simulink model "LKA_Controller"  (R2026a)
settings: Solver=FixedStepDiscrete  StopTime=inf  FixedStep=LKA.Ts
undefined symbols (not defined in the file): DiscIntNeverNeededParam, LKA
libraries: simulink x6, sl_discontinuities x2
Description:
  | Lane Keeping Assist: lane perception (validation, centre fusion, Kalman tracker), supervisor FSM, lane departure warning, pure pursuit / Stanley 2025 / MPC lateral controllers, a_y and jerk limited curvature command, steering actuator manager, turning radius.
settings Model: Creator=rithv  LastModifiedBy=rithv
settings DebuggingCC: AlgebraicLoopMsg=error
settings ModelReferenceCC: ModelReferenceNumInstancesAllowed=Single
settings GRTTargetCC: SubcomponentCodeInterfacePackaging=Nonreusable function

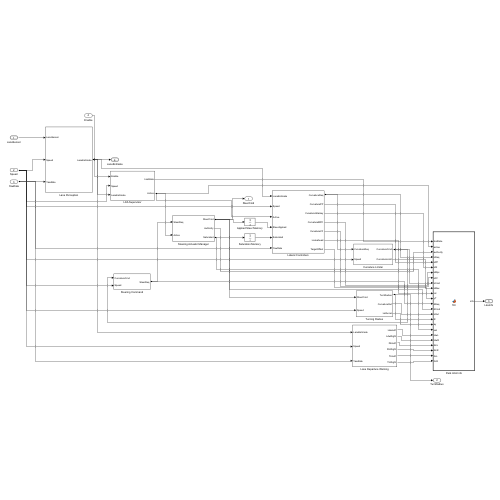
[thumbnail: Simulink's stored preview of the top-level diagram]
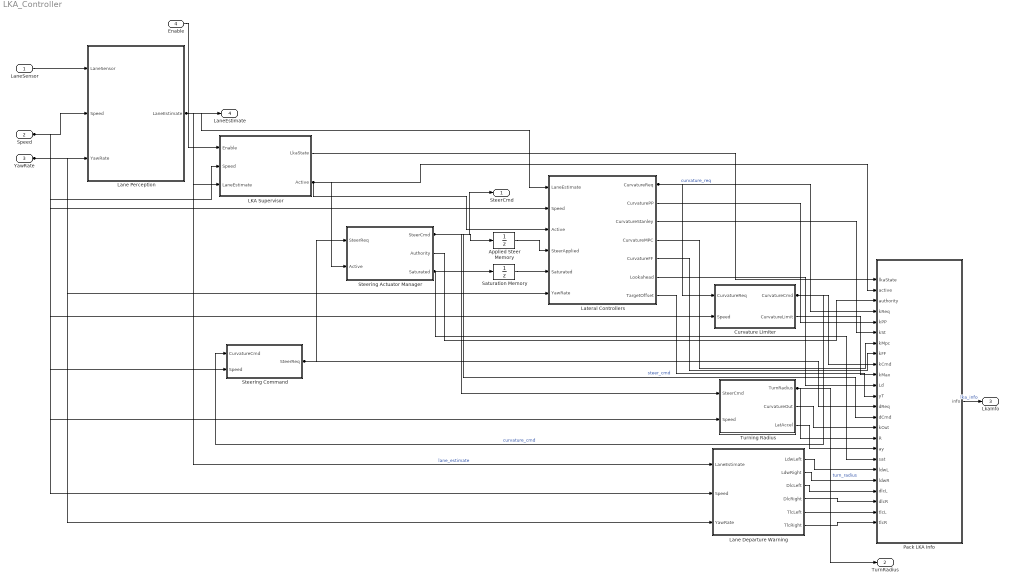
== system LKA_Controller ==
  LaneSensor : Inport  OutDataTypeStr=Bus: LaneSensorBus  SampleTime=LKA.Ts  BusOutputAsStruct=on
  Speed : Inport  Port=2  OutDataTypeStr=double  SampleTime=LKA.Ts
  YawRate : Inport  Port=3  OutDataTypeStr=double  SampleTime=LKA.Ts
  Enable : Inport  Port=4  OutDataTypeStr=boolean  SampleTime=LKA.Ts
  Applied Steer Memory : UnitDelay  SampleTime=-1
  Curvature Limiter : Subsystem
  LKA Supervisor : Subsystem
  Lane Departure Warning : Subsystem
  Lane Perception : Subsystem
  Lateral Controllers : Subsystem
  Pack LKA Info : MATLAB Function  TreatAsAtomicUnit=on
  Saturation Memory : UnitDelay  SampleTime=-1
  Steering Actuator Manager : Subsystem
  Steering Command : Subsystem
  Turning Radius : Subsystem
  SteerCmd : Outport  OutDataTypeStr=double
  TurnRadius : Outport  Port=2  OutDataTypeStr=double
  LkaInfo : Outport  Port=3  OutDataTypeStr=Bus: LkaInfoBus  BusOutputAsStruct=on
  LaneEstimate : Outport  Port=4  OutDataTypeStr=Bus: LaneEstimateBus  BusOutputAsStruct=on
  wires:
  Turning Radius/1(TurnRadius) -> TurnRadius/1, Pack LKA Info/16(R)  "turn_radius"
  Steering Command/1(SteerReq) -> Pack LKA Info/13(dReq), Steering Actuator Manager/1(SteerReq)
  Lane Departure Warning/2(LdwRight) -> Pack LKA Info/20(ldwR)
  LaneSensor/1 -> Lane Perception/1(LaneSensor)
  Steering Actuator Manager/1(SteerCmd) -> Turning Radius/1(SteerCmd), Pack LKA Info/14(dCmd), Applied Steer Memory/1, SteerCmd/1  "steer_cmd"
  Speed/1 -> LKA Supervisor/2(Speed), Lateral Controllers/2(Speed), Curvature Limiter/2(Speed), Steering Command/2(Speed), Turning Radius/2(Speed), Lane Perception/2(Speed), Lane Departure Warning/2(Speed)
  Enable/1 -> LKA Supervisor/1(Enable)
  Lane Departure Warning/5(TlcLeft) -> Pack LKA Info/23(tlcL)
  Lateral Controllers/5(CurvatureFF) -> Pack LKA Info/8(kFF)
  YawRate/1 -> Lateral Controllers/6(YawRate), Lane Perception/3(YawRate), Lane Departure Warning/3(YawRate)
  Lateral Controllers/2(CurvaturePP) -> Pack LKA Info/5(kPP)
  Saturation Memory/1 -> Lateral Controllers/5(Saturated)
  LKA Supervisor/1(LkaState) -> Pack LKA Info/1(lkaState)
  Lane Perception/1(LaneEstimate) -> Lateral Controllers/1(LaneEstimate), LKA Supervisor/3(LaneEstimate), LaneEstimate/1, Lane Departure Warning/1(LaneEstimate)  "lane_estimate"
  LKA Supervisor/2(Active) -> Lateral Controllers/3(Active), Pack LKA Info/2(active), Steering Actuator Manager/2(Active)
  Steering Actuator Manager/2(Authority) -> Pack LKA Info/3(authority)
  Steering Actuator Manager/3(Saturated) -> Pack LKA Info/18(sat), Saturation Memory/1
  Applied Steer Memory/1 -> Lateral Controllers/4(SteerApplied)
  Lateral Controllers/1(CurvatureReq) -> Curvature Limiter/1(CurvatureReq), Pack LKA Info/4(kReq)  "curvature_req"
  Lateral Controllers/3(CurvatureStanley) -> Pack LKA Info/6(kSt)
  Lateral Controllers/4(CurvatureMPC) -> Pack LKA Info/7(kMpc)
  Lateral Controllers/6(Lookahead) -> Pack LKA Info/11(Ld)
  Lateral Controllers/7(TargetOffset) -> Pack LKA Info/12(yT)
  Curvature Limiter/1(CurvatureCmd) -> Steering Command/1(CurvatureCmd), Pack LKA Info/9(kCmd)  "curvature_cmd"
  Curvature Limiter/2(CurvatureLimit) -> Pack LKA Info/10(kMax)
  Turning Radius/2(CurvatureOut) -> Pack LKA Info/15(kOut)
  Turning Radius/3(LatAccel) -> Pack LKA Info/17(ay)
  Lane Departure Warning/6(TlcRight) -> Pack LKA Info/24(tlcR)
  Lane Departure Warning/1(LdwLeft) -> Pack LKA Info/19(ldwL)
  Lane Departure Warning/3(DlcLeft) -> Pack LKA Info/21(dlcL)
  Lane Departure Warning/4(DlcRight) -> Pack LKA Info/22(dlcR)
  Pack LKA Info/1(info) -> LkaInfo/1  "lka_info"

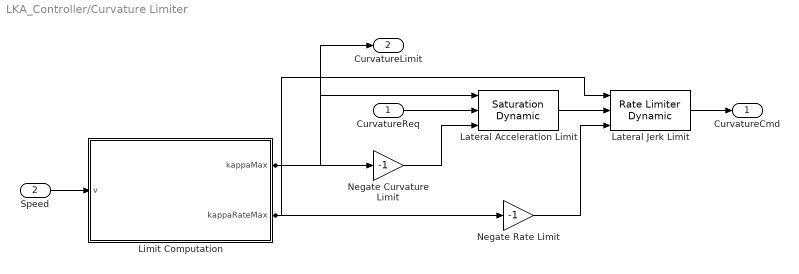
== system LKA_Controller/Curvature Limiter ==
  CurvatureReq : Inport
  Speed : Inport  Port=2
  Lateral Acceleration Limit : sl_discontinuities/Saturation Dynamic  OutMin=[]  OutMax=[]  OutDataTypeStr=Inherit: Same as second input  OutDataType=fixdt(1, 16)  OutScaling=2^-10  DoSatur=off
      settings: LibrarySourceBlock=|
      | simulink/Discontinuities/Saturation
      | Dynamic
  Lateral Jerk Limit : sl_discontinuities/Rate Limiter Dynamic
      settings: LibrarySourceBlock=|
      | simulink/Discontinuities/Rate Limiter
      | Dynamic
  Limit Computation : MATLAB Function  TreatAsAtomicUnit=on
  Negate Curvature Limit : Gain  Gain=-1
  Negate Rate Limit : Gain  Gain=-1
  CurvatureCmd : Outport
  CurvatureLimit : Outport  Port=2
  wires:
  Lateral Acceleration Limit/1 -> Lateral Jerk Limit/2
  Speed/1 -> Limit Computation/1(v)
  Negate Rate Limit/1 -> Lateral Jerk Limit/3
  CurvatureReq/1 -> Lateral Acceleration Limit/2
  Limit Computation/1(kappaMax) -> Negate Curvature Limit/1, Lateral Acceleration Limit/1, CurvatureLimit/1
  Limit Computation/2(kappaRateMax) -> Lateral Jerk Limit/1, Negate Rate Limit/1
  Lateral Jerk Limit/1 -> CurvatureCmd/1
  Negate Curvature Limit/1 -> Lateral Acceleration Limit/3

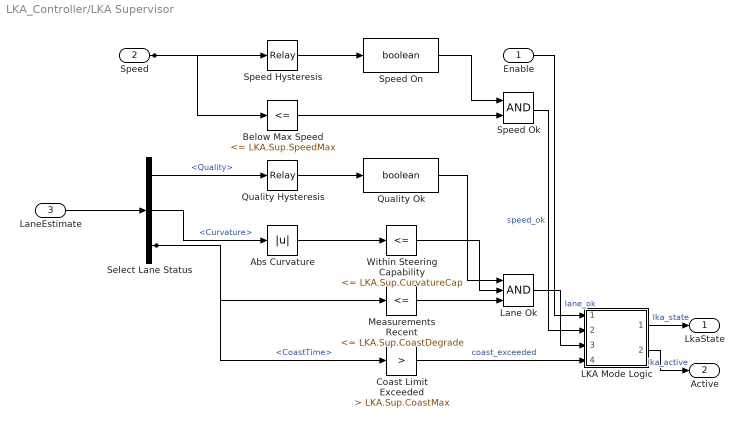
== system LKA_Controller/LKA Supervisor ==
  Enable : Inport
  Speed : Inport  Port=2
  LaneEstimate : Inport  Port=3
  Abs Curvature : Abs  SaturateOnIntegerOverflow=off
  Below Max Speed : simulink/Logic and Bit Operations/Compare To Constant  relop=<=  const=LKA.Sup.SpeedMax  OutDataTypeStr=boolean
  Coast Limit Exceeded : simulink/Logic and Bit Operations/Compare To Constant  relop=>  const=LKA.Sup.CoastMax  OutDataTypeStr=boolean
  LKA Mode Logic : Stateflow chart  TreatAsAtomicUnit=on
  Lane Ok : Logic  Inputs=3  AllPortsSameDT=off  OutDataTypeStr=boolean
  Measurements Recent : simulink/Logic and Bit Operations/Compare To Constant  relop=<=  const=LKA.Sup.CoastDegrade  OutDataTypeStr=boolean
  Quality Hysteresis : Relay  OnSwitchValue=LKA.Sup.QualityOn  OffSwitchValue=LKA.Sup.QualityOff
  Quality Ok : DataTypeConversion  OutDataTypeStr=boolean  SaturateOnIntegerOverflow=off  RndMeth=Floor
  Select Lane Status : BusSelector  OutputSignals=Quality,Curvature,CoastTime
  Speed Hysteresis : Relay  OnSwitchValue=LKA.Sup.SpeedOn  OffSwitchValue=LKA.Sup.SpeedOff
  Speed Ok : Logic  AllPortsSameDT=off  OutDataTypeStr=boolean
  Speed On : DataTypeConversion  OutDataTypeStr=boolean  SaturateOnIntegerOverflow=off  RndMeth=Floor
  Within Steering Capability : simulink/Logic and Bit Operations/Compare To Constant  relop=<=  const=LKA.Sup.CurvatureCap  OutDataTypeStr=boolean
  LkaState : Outport
  Active : Outport  Port=2
  wires:
  LKA Mode Logic/1(lkaState) -> LkaState/1  "lka_state"
  LaneEstimate/1 -> Select Lane Status/1
  Speed/1 -> Speed Hysteresis/1, Below Max Speed/1
  Select Lane Status/2 -> Abs Curvature/1  "<Curvature>"
  Speed Ok/1 -> LKA Mode Logic/2(speedOk)  "speed_ok"
  Select Lane Status/1 -> Quality Hysteresis/1  "<Quality>"
  Enable/1 -> LKA Mode Logic/1(enable)
  Quality Hysteresis/1 -> Quality Ok/1
  Select Lane Status/3 -> Measurements Recent/1, Coast Limit Exceeded/1  "<CoastTime>"
  Speed Hysteresis/1 -> Speed On/1
  Below Max Speed/1 -> Speed Ok/2
  Abs Curvature/1 -> Within Steering Capability/1
  Speed On/1 -> Speed Ok/1
  Quality Ok/1 -> Lane Ok/1
  Within Steering Capability/1 -> Lane Ok/2
  Measurements Recent/1 -> Lane Ok/3
  Coast Limit Exceeded/1 -> LKA Mode Logic/4(coastExceeded)  "coast_exceeded"
  Lane Ok/1 -> LKA Mode Logic/3(laneOk)  "lane_ok"
  LKA Mode Logic/2(active) -> Active/1  "lka_active"

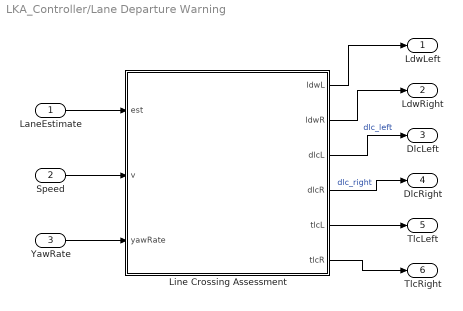
== system LKA_Controller/Lane Departure Warning ==
  LaneEstimate : Inport
  Speed : Inport  Port=2
  YawRate : Inport  Port=3
  Line Crossing Assessment : MATLAB Function  TreatAsAtomicUnit=on
  LdwLeft : Outport
  LdwRight : Outport  Port=2
  DlcLeft : Outport  Port=3
  DlcRight : Outport  Port=4
  TlcLeft : Outport  Port=5
  TlcRight : Outport  Port=6
  wires:
  Line Crossing Assessment/4(dlcR) -> DlcRight/1  "dlc_right"
  YawRate/1 -> Line Crossing Assessment/3(yawRate)
  LaneEstimate/1 -> Line Crossing Assessment/1(est)
  Line Crossing Assessment/2(ldwR) -> LdwRight/1
  Speed/1 -> Line Crossing Assessment/2(v)
  Line Crossing Assessment/1(ldwL) -> LdwLeft/1
  Line Crossing Assessment/5(tlcL) -> TlcLeft/1
  Line Crossing Assessment/3(dlcL) -> DlcLeft/1  "dlc_left"
  Line Crossing Assessment/6(tlcR) -> TlcRight/1

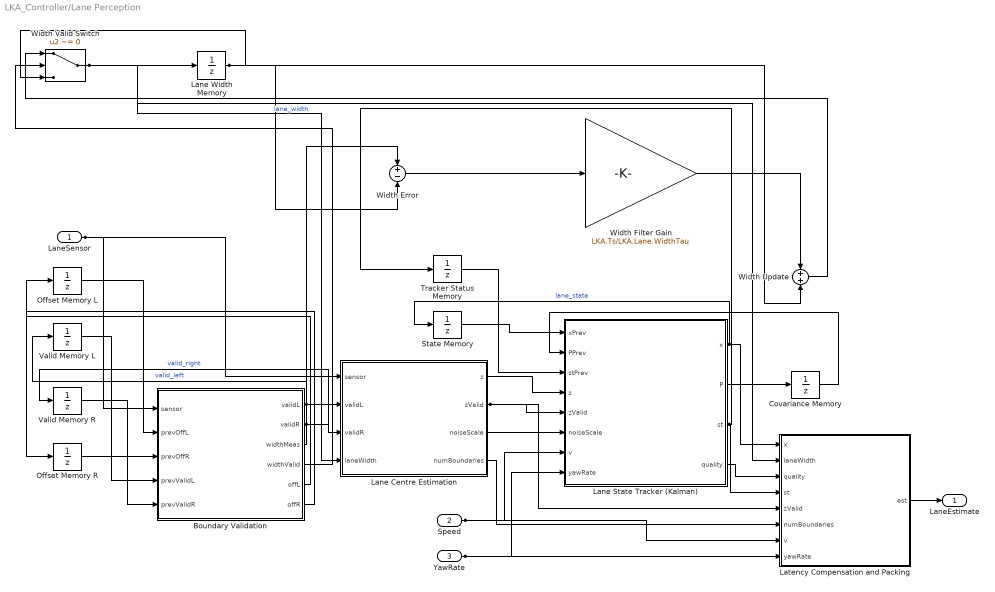
== system LKA_Controller/Lane Perception ==
  LaneSensor : Inport
  Speed : Inport  Port=2
  YawRate : Inport  Port=3
  Boundary Validation : MATLAB Function  TreatAsAtomicUnit=on
  Covariance Memory : UnitDelay  InitialCondition=eye(4)  SampleTime=-1
  Lane Centre Estimation : MATLAB Function  TreatAsAtomicUnit=on
  Lane State Tracker (Kalman) : MATLAB Function  TreatAsAtomicUnit=on
  Lane Width Memory : UnitDelay  InitialCondition=LKA.Lane.WidthNominal  SampleTime=-1
  Latency Compensation and Packing : MATLAB Function  TreatAsAtomicUnit=on
  Offset Memory L : UnitDelay  SampleTime=-1
  Offset Memory R : UnitDelay  SampleTime=-1
  State Memory : UnitDelay  InitialCondition=zeros(4,1)  SampleTime=-1
  Tracker Status Memory : UnitDelay  InitialCondition=zeros(3,1)  SampleTime=-1
  Valid Memory L : UnitDelay  SampleTime=-1
  Valid Memory R : UnitDelay  SampleTime=-1
  Width Error : Sum  Inputs=+-
  Width Filter Gain : Gain  Gain=LKA.Ts/LKA.Lane.WidthTau
  Width Update : Sum
  Width Valid Switch : Switch  Criteria=u2 ~= 0  SaturateOnIntegerOverflow=off  InputSameDT=off
  LaneEstimate : Outport
  wires:
  Valid Memory L/1 -> Boundary Validation/4(prevValidL)
  LaneSensor/1 -> Boundary Validation/1(sensor), Lane Centre Estimation/1(sensor)
  Width Valid Switch/1 -> Lane Centre Estimation/4(laneWidth), Latency Compensation and Packing/2(laneWidth), Lane Width Memory/1  "lane_width"
  Offset Memory L/1 -> Boundary Validation/2(prevOffL)
  Boundary Validation/1(validL) -> Valid Memory L/1, Lane Centre Estimation/2(validL)  "valid_left"
  Offset Memory R/1 -> Boundary Validation/3(prevOffR)
  Valid Memory R/1 -> Boundary Validation/5(prevValidR)
  Lane Width Memory/1 -> Width Valid Switch/3, Width Update/2, Width Error/2
  Boundary Validation/2(validR) -> Valid Memory R/1, Lane Centre Estimation/3(validR)  "valid_right"
  Lane State Tracker (Kalman)/1(x) -> State Memory/1, Latency Compensation and Packing/1(x)  "lane_state"
  Boundary Validation/3(widthMeas) -> Width Error/1
  Covariance Memory/1 -> Lane State Tracker (Kalman)/2(PPrev)
  Boundary Validation/4(widthValid) -> Width Valid Switch/2
  Boundary Validation/5(offL) -> Offset Memory L/1
  Lane Centre Estimation/3(noiseScale) -> Lane State Tracker (Kalman)/6(noiseScale)
  Boundary Validation/6(offR) -> Offset Memory R/1
  Width Error/1 -> Width Filter Gain/1
  Lane Centre Estimation/1(z) -> Lane State Tracker (Kalman)/4(z)
  Tracker Status Memory/1 -> Lane State Tracker (Kalman)/3(stPrev)
  Lane State Tracker (Kalman)/2(P) -> Covariance Memory/1
  State Memory/1 -> Lane State Tracker (Kalman)/1(xPrev)
  Lane Centre Estimation/2(zValid) -> Latency Compensation and Packing/5(zValid), Lane State Tracker (Kalman)/5(zValid)
  Lane Centre Estimation/4(numBoundaries) -> Latency Compensation and Packing/6(numBoundaries)
  Speed/1 -> Latency Compensation and Packing/7(v), Lane State Tracker (Kalman)/7(v)
  YawRate/1 -> Latency Compensation and Packing/8(yawRate), Lane State Tracker (Kalman)/8(yawRate)
  Width Filter Gain/1 -> Width Update/1
  Lane State Tracker (Kalman)/3(st) -> Tracker Status Memory/1, Latency Compensation and Packing/4(st)
  Lane State Tracker (Kalman)/4(quality) -> Latency Compensation and Packing/3(quality)
  Width Update/1 -> Width Valid Switch/1
  Latency Compensation and Packing/1(est) -> LaneEstimate/1

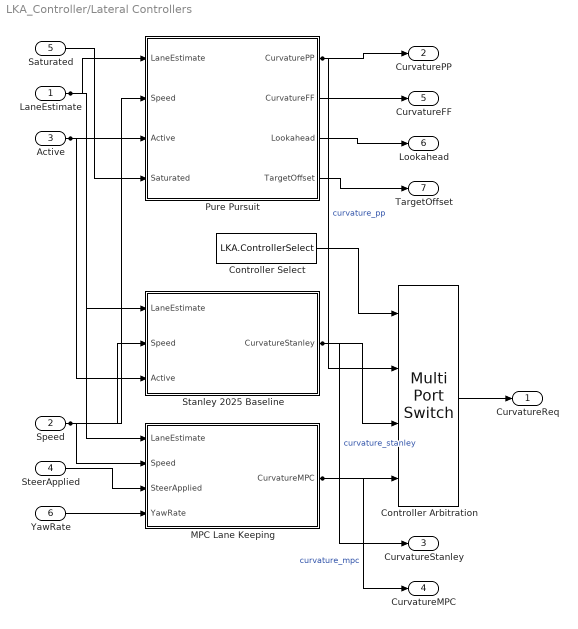
== system LKA_Controller/Lateral Controllers ==
  LaneEstimate : Inport
  Speed : Inport  Port=2
  Active : Inport  Port=3
  SteerApplied : Inport  Port=4
  Saturated : Inport  Port=5
  YawRate : Inport  Port=6
  Controller Arbitration : MultiPortSwitch  SaturateOnIntegerOverflow=off  InputSameDT=off
  Controller Select : Constant  Value=LKA.ControllerSelect
  MPC Lane Keeping : Subsystem
  Pure Pursuit : Subsystem
  Stanley 2025 Baseline : Subsystem
  CurvatureReq : Outport
  CurvaturePP : Outport  Port=2
  CurvatureStanley : Outport  Port=3
  CurvatureMPC : Outport  Port=4
  CurvatureFF : Outport  Port=5
  Lookahead : Outport  Port=6
  TargetOffset : Outport  Port=7
  wires:
  Pure Pursuit/1(CurvaturePP) -> Controller Arbitration/2, CurvaturePP/1  "curvature_pp"
  Saturated/1 -> Pure Pursuit/4(Saturated)
  LaneEstimate/1 -> Pure Pursuit/1(LaneEstimate), MPC Lane Keeping/1(LaneEstimate), Stanley 2025 Baseline/1(LaneEstimate)
  Active/1 -> Pure Pursuit/3(Active), Stanley 2025 Baseline/3(Active)
  YawRate/1 -> MPC Lane Keeping/4(YawRate)
  Speed/1 -> Stanley 2025 Baseline/2(Speed), MPC Lane Keeping/2(Speed), Pure Pursuit/2(Speed)
  SteerApplied/1 -> MPC Lane Keeping/3(SteerApplied)
  Pure Pursuit/2(CurvatureFF) -> CurvatureFF/1
  MPC Lane Keeping/1(CurvatureMPC) -> Controller Arbitration/4, CurvatureMPC/1  "curvature_mpc"
  Stanley 2025 Baseline/1(CurvatureStanley) -> Controller Arbitration/3, CurvatureStanley/1  "curvature_stanley"
  Pure Pursuit/3(Lookahead) -> Lookahead/1
  Pure Pursuit/4(TargetOffset) -> TargetOffset/1
  Controller Select/1 -> Controller Arbitration/1
  Controller Arbitration/1 -> CurvatureReq/1

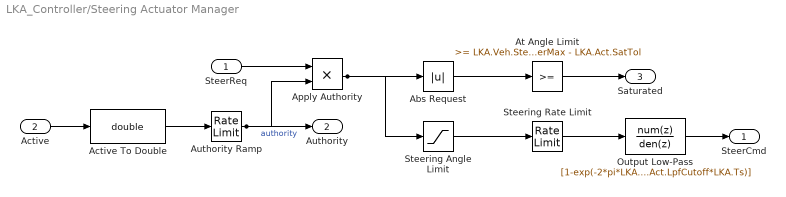
== system LKA_Controller/Steering Actuator Manager ==
  SteerReq : Inport
  Active : Inport  Port=2
  Abs Request : Abs  SaturateOnIntegerOverflow=off
  Active To Double : DataTypeConversion  OutDataTypeStr=double  SaturateOnIntegerOverflow=off  RndMeth=Floor
  Apply Authority : Product
  At Angle Limit : simulink/Logic and Bit Operations/Compare To Constant  relop=>=  const=LKA.Veh.SteerMax - LKA.Act.SatTol  OutDataTypeStr=boolean
  Authority Ramp : RateLimiter  RisingSlewLimit=1/LKA.Act.RampTime  FallingSlewLimit=-1/LKA.Act.RampTime  SampleTimeMode=inherited
  Output Low-Pass : DiscreteTransferFcn  Numerator=[1-exp(-2*pi*LKA.Act.LpfCutoff*LKA.Ts)]  Denominator=[1 -exp(-2*pi*LKA.Act.LpfCutoff*LKA.Ts)]
  Steering Angle Limit : Saturate  UpperLimit=LKA.Veh.SteerMax  LowerLimit=-LKA.Veh.SteerMax
  Steering Rate Limit : RateLimiter  RisingSlewLimit=LKA.Veh.SteerRateMax  FallingSlewLimit=-LKA.Veh.SteerRateMax  SampleTimeMode=inherited
  SteerCmd : Outport
  Authority : Outport  Port=2
  Saturated : Outport  Port=3
  wires:
  Steering Angle Limit/1 -> Steering Rate Limit/1
  Active/1 -> Active To Double/1
  Authority Ramp/1 -> Apply Authority/2, Authority/1  "authority"
  Active To Double/1 -> Authority Ramp/1
  At Angle Limit/1 -> Saturated/1
  SteerReq/1 -> Apply Authority/1
  Apply Authority/1 -> Steering Angle Limit/1, Abs Request/1
  Abs Request/1 -> At Angle Limit/1
  Steering Rate Limit/1 -> Output Low-Pass/1
  Output Low-Pass/1 -> SteerCmd/1

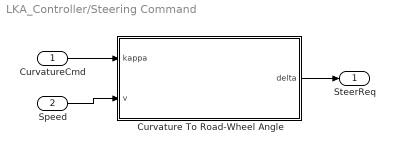
== system LKA_Controller/Steering Command ==
  CurvatureCmd : Inport
  Speed : Inport  Port=2
  Curvature To Road-Wheel Angle : MATLAB Function  TreatAsAtomicUnit=on
  SteerReq : Outport
  wires:
  CurvatureCmd/1 -> Curvature To Road-Wheel Angle/1(kappa)
  Speed/1 -> Curvature To Road-Wheel Angle/2(v)
  Curvature To Road-Wheel Angle/1(delta) -> SteerReq/1

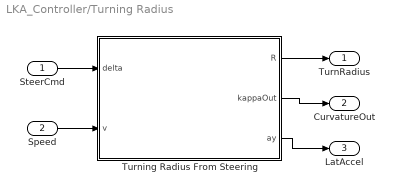
== system LKA_Controller/Turning Radius ==
  SteerCmd : Inport
  Speed : Inport  Port=2
  Turning Radius From Steering : MATLAB Function  TreatAsAtomicUnit=on
  TurnRadius : Outport
  CurvatureOut : Outport  Port=2
  LatAccel : Outport  Port=3
  wires:
  Turning Radius From Steering/2(kappaOut) -> CurvatureOut/1
  SteerCmd/1 -> Turning Radius From Steering/1(delta)
  Turning Radius From Steering/3(ay) -> LatAccel/1
  Speed/1 -> Turning Radius From Steering/2(v)
  Turning Radius From Steering/1(R) -> TurnRadius/1

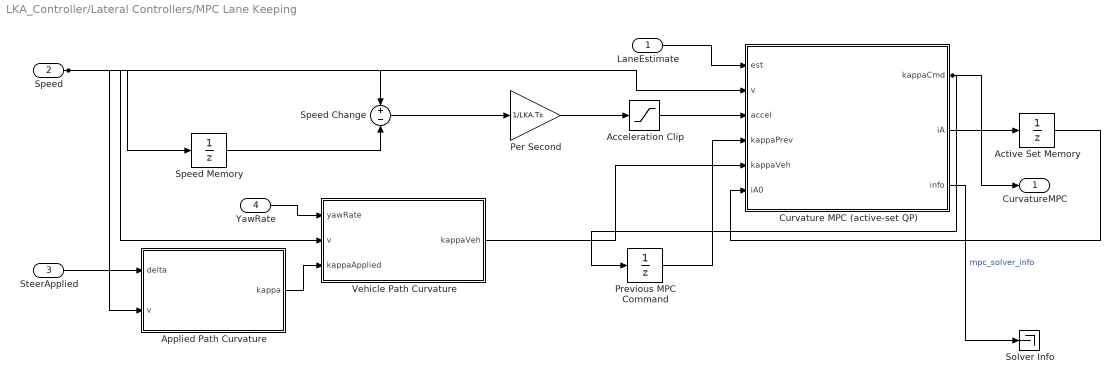
== system LKA_Controller/Lateral Controllers/MPC Lane Keeping ==
  LaneEstimate : Inport
  Speed : Inport  Port=2
  SteerApplied : Inport  Port=3
  YawRate : Inport  Port=4
  Acceleration Clip : Saturate  UpperLimit=LKA.Mpc.AccelMax  LowerLimit=-LKA.Mpc.AccelMax
  Active Set Memory : UnitDelay  InitialCondition=false(120,1)  SampleTime=-1
  Applied Path Curvature : MATLAB Function  TreatAsAtomicUnit=on
  Curvature MPC (active-set QP) : MATLAB Function  TreatAsAtomicUnit=on
  Per Second : Gain  Gain=1/LKA.Ts
  Previous MPC Command : UnitDelay  SampleTime=-1
  Solver Info : Terminator
  Speed Change : Sum  Inputs=+-
  Speed Memory : UnitDelay  SampleTime=-1
  Vehicle Path Curvature : MATLAB Function  TreatAsAtomicUnit=on
  CurvatureMPC : Outport
  wires:
  Speed/1 -> Speed Change/1, Curvature MPC (active-set QP)/2(v), Vehicle Path Curvature/2(v), Speed Memory/1, Applied Path Curvature/2(v)
  Per Second/1 -> Acceleration Clip/1
  SteerApplied/1 -> Applied Path Curvature/1(delta)
  Speed Change/1 -> Per Second/1
  LaneEstimate/1 -> Curvature MPC (active-set QP)/1(est)
  Applied Path Curvature/1(kappa) -> Vehicle Path Curvature/3(kappaApplied)
  Speed Memory/1 -> Speed Change/2
  YawRate/1 -> Vehicle Path Curvature/1(yawRate)
  Previous MPC Command/1 -> Curvature MPC (active-set QP)/4(kappaPrev)
  Vehicle Path Curvature/1(kappaVeh) -> Curvature MPC (active-set QP)/5(kappaVeh)
  Acceleration Clip/1 -> Curvature MPC (active-set QP)/3(accel)
  Curvature MPC (active-set QP)/1(kappaCmd) -> Previous MPC Command/1, CurvatureMPC/1
  Curvature MPC (active-set QP)/2(iA) -> Active Set Memory/1
  Curvature MPC (active-set QP)/3(info) -> Solver Info/1  "mpc_solver_info"
  Active Set Memory/1 -> Curvature MPC (active-set QP)/6(iA0)

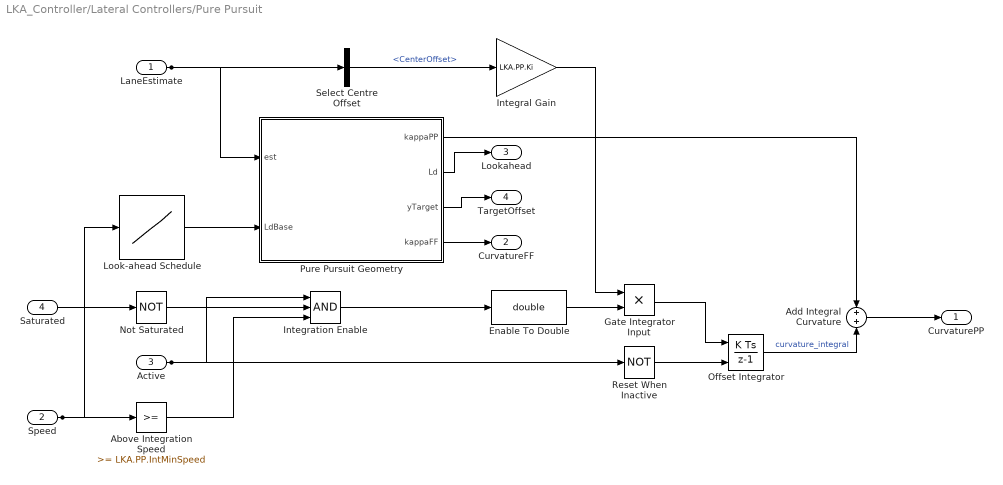
== system LKA_Controller/Lateral Controllers/Pure Pursuit ==
  LaneEstimate : Inport
  Speed : Inport  Port=2
  Active : Inport  Port=3
  Saturated : Inport  Port=4
  Above Integration Speed : simulink/Logic and Bit Operations/Compare To Constant  relop=>=  const=LKA.PP.IntMinSpeed  OutDataTypeStr=boolean
  Add Integral Curvature : Sum
  Enable To Double : DataTypeConversion  OutDataTypeStr=double  SaturateOnIntegerOverflow=off  RndMeth=Floor
  Gate Integrator Input : Product
  Integral Gain : Gain  Gain=LKA.PP.Ki
  Integration Enable : Logic  Inputs=3  AllPortsSameDT=off  OutDataTypeStr=boolean
  Look-ahead Schedule : Lookup_n-D  NumberOfTableDimensions=1  BreakpointsForDimension1=LKA.PP.LdSpeed  Table=LKA.PP.LdBase  ExtrapMethod=Clip  InternalRulePriority=Speed  RndMeth=Simplest
  Not Saturated : Logic  Operator=NOT  Inputs=1  AllPortsSameDT=off  OutDataTypeStr=boolean
  Offset Integrator : DiscreteIntegrator  ExternalReset=level  SampleTime=-1  LimitOutput=on  UpperSaturationLimit=LKA.PP.IntLimit  LowerSaturationLimit=-LKA.PP.IntLimit  ICPrevOutput=DiscIntNeverNeededParam  ICPrevScaledInput=DiscIntNeverNeededParam
  Pure Pursuit Geometry : MATLAB Function  TreatAsAtomicUnit=on
  Reset When Inactive : Logic  Operator=NOT  Inputs=1  AllPortsSameDT=off  OutDataTypeStr=boolean
  Select Centre Offset : BusSelector  OutputSignals=CenterOffset
  CurvaturePP : Outport
  CurvatureFF : Outport  Port=2
  Lookahead : Outport  Port=3
  TargetOffset : Outport  Port=4
  wires:
  Active/1 -> Reset When Inactive/1, Integration Enable/1
  Look-ahead Schedule/1 -> Pure Pursuit Geometry/2(LdBase)
  Saturated/1 -> Not Saturated/1
  Reset When Inactive/1 -> Offset Integrator/2
  Above Integration Speed/1 -> Integration Enable/3
  Enable To Double/1 -> Gate Integrator Input/2
  Speed/1 -> Look-ahead Schedule/1, Above Integration Speed/1
  Not Saturated/1 -> Integration Enable/2
  LaneEstimate/1 -> Pure Pursuit Geometry/1(est), Select Centre Offset/1
  Select Centre Offset/1 -> Integral Gain/1  "<CenterOffset>"
  Pure Pursuit Geometry/1(kappaPP) -> Add Integral Curvature/1
  Pure Pursuit Geometry/2(Ld) -> Lookahead/1
  Pure Pursuit Geometry/3(yTarget) -> TargetOffset/1
  Pure Pursuit Geometry/4(kappaFF) -> CurvatureFF/1
  Add Integral Curvature/1 -> CurvaturePP/1
  Integration Enable/1 -> Enable To Double/1
  Integral Gain/1 -> Gate Integrator Input/1
  Gate Integrator Input/1 -> Offset Integrator/1
  Offset Integrator/1 -> Add Integral Curvature/2  "curvature_integral"

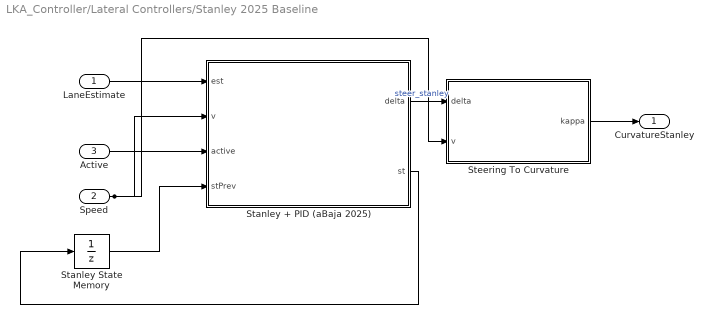
== system LKA_Controller/Lateral Controllers/Stanley 2025 Baseline ==
  LaneEstimate : Inport
  Speed : Inport  Port=2
  Active : Inport  Port=3
  Stanley + PID (aBaja 2025) : MATLAB Function  TreatAsAtomicUnit=on
  Stanley State Memory : UnitDelay  InitialCondition=zeros(6,1)  SampleTime=-1
  Steering To Curvature : MATLAB Function  TreatAsAtomicUnit=on
  CurvatureStanley : Outport
  wires:
  LaneEstimate/1 -> Stanley + PID (aBaja 2025)/1(est)
  Active/1 -> Stanley + PID (aBaja 2025)/3(active)
  Steering To Curvature/1(kappa) -> CurvatureStanley/1
  Stanley + PID (aBaja 2025)/1(delta) -> Steering To Curvature/1(delta)  "steer_stanley"
  Speed/1 -> Steering To Curvature/2(v), Stanley + PID (aBaja 2025)/2(v)
  Stanley State Memory/1 -> Stanley + PID (aBaja 2025)/4(stPrev)
  Stanley + PID (aBaja 2025)/2(st) -> Stanley State Memory/1

== matlab function LKA_Controller/Lane Departure Warning/Line Crossing Assessment ==
  data: est input Bus: LaneEstimateBus; ldwL output; v input; yawRate input; ldwR output; dlcL output; dlcR output; tlcL output; tlcR output; LKA parameter
function [ldwL, ldwR, dlcL, dlcR, tlcL, tlcR] = fcn(est, v, yawRate, LKA)
% Distance / time to line crossing of the tyre edges and LDW (see lka_lane_departure.m)
[ldwL, ldwR, dlcL, dlcR, tlcL, tlcR] = lka_lane_departure(est, v, yawRate, est.Quality, LKA.Veh, LKA.Lane, LKA.Ldw);

== matlab function LKA_Controller/Lateral Controllers/Pure Pursuit/Pure Pursuit Geometry ==
  data: est input Bus: LaneEstimateBus; kappaPP output; LdBase input; Ld output; yTarget output; kappaFF output; LKA parameter
function [kappaPP, Ld, yTarget, kappaFF] = fcn(est, LdBase, LKA)
% Arc from the rear axle to the lane-centre point Ld ahead: kappa = 2*yT/(Ld^2 + yT^2)
[kappaPP, Ld, yTarget, kappaFF] = lka_pure_pursuit(est, LdBase, LKA.PP);

== matlab function LKA_Controller/Lateral Controllers/Stanley 2025 Baseline/Stanley + PID (aBaja 2025) ==
  data: est input Bus: LaneEstimateBus; delta output double size=1; v input; active input; stPrev input; st output double size=[6 1]; LKA parameter
function [delta, st] = fcn(est, v, active, stPrev, LKA)
% 2025 lka.py control law, errors taken from the vehicle-frame lane estimate
[delta, st] = lka_stanley_2025(est, v, active, stPrev, LKA.Ts, LKA.St);

== matlab function LKA_Controller/Lateral Controllers/Stanley 2025 Baseline/Steering To Curvature ==
  data: delta input; kappa output; v input; LKA parameter
function kappa = fcn(delta, v, LKA)
% kappa = tan(delta) / (L + K_us*v^2)
kappa = lka_steer_to_curvature(delta, v, LKA.Veh);

== matlab function LKA_Controller/Lateral Controllers/MPC Lane Keeping/Applied Path Curvature ==
  data: delta input; kappa output; v input; LKA parameter
function kappa = fcn(delta, v, LKA)
% kappa = tan(delta) / (L + K_us*v^2)
kappa = lka_steer_to_curvature(delta, v, LKA.Veh);

== matlab function LKA_Controller/Lateral Controllers/MPC Lane Keeping/Vehicle Path Curvature ==
  data: yawRate input; kappaVeh output; v input; kappaApplied input
function kappaVeh = fcn(yawRate, v, kappaApplied)
% Measured path curvature of the rear axle, r/v (falls back to the steering command at low speed)
if v > 1
    kappaVeh = yawRate / v;
else
    kappaVeh = kappaApplied;
end

== matlab function LKA_Controller/Lateral Controllers/MPC Lane Keeping/Curvature MPC (active-set QP) ==
  data: est input Bus: LaneEstimateBus; kappaCmd output double size=1; v input; accel input; kappaPrev input; kappaVeh input; iA0 input; iA output boolean size=[120 1]; info output double size=[2 1]; LKA parameter
function [kappaCmd, iA, info] = fcn(est, v, accel, kappaPrev, kappaVeh, iA0, LKA)
% LTV lane-error MPC: model e_y, e_psi, kappa_v along the predicted speed profile;
% preview kappa_road; |kappa| and |dkappa| constrained per step
[kappaCmd, iA, info] = lka_mpc_curvature(est, v, accel, kappaPrev, kappaVeh, iA0, ...
    LKA.Mpc, LKA.Veh, LKA.Lim, LKA.Ts);

== matlab function LKA_Controller/Curvature Limiter/Limit Computation ==
  data: v input; kappaMax output; kappaRateMax output; LKA parameter
function [kappaMax, kappaRateMax] = fcn(v, LKA)
% |kappa| <= a_y,max/v^2 and steering-angle limit; |dkappa/dt| <= jerk_max/v^2 and steering-rate limit
[kappaMax, kappaRateMax] = lka_curvature_limits(v, LKA.Veh, LKA.Lim);

== matlab function LKA_Controller/Steering Command/Curvature To Road-Wheel Angle ==
  data: kappa input; delta output; v input; LKA parameter
function delta = fcn(kappa, v, LKA)
% Single-track steady-state steering: delta = atan(kappa*(L + K_us*v^2))
delta = lka_curvature_to_steer(kappa, v, LKA.Veh);

== matlab function LKA_Controller/Turning Radius/Turning Radius From Steering ==
  data: delta input; R output; v input; kappaOut output; ay output; LKA parameter
function [R, kappaOut, ay] = fcn(delta, v, LKA)
% Path curvature and turning radius produced by the commanded road-wheel angle
kappaOut = lka_steer_to_curvature(delta, v, LKA.Veh);
Rmax = LKA.Out.RadiusMax;
if abs(kappaOut) > 1/Rmax
    R = 1/kappaOut;
elseif kappaOut >= 0
    R = Rmax;
else
    R = -Rmax;
end
ay = v^2*kappaOut;

== matlab function LKA_Controller/Pack LKA Info ==
  data: lkaState input; info output Bus: LkaInfoBus; active input; authority input; kReq input; kPP input; kSt input; kMpc input; kFF input; kCmd input; kMax input; Ld input; yT input; dReq input; dCmd input; kOut input; R input; ay input; sat input; ldwL input; ldwR input; dlcL input; dlcR input; tlcL input; tlcR input; LKA parameter
function info = fcn(lkaState, active, authority, kReq, kPP, kSt, kMpc, kFF, kCmd, kMax, Ld, yT, ...
    dReq, dCmd, kOut, R, ay, sat, ldwL, ldwR, dlcL, dlcR, tlcL, tlcR, LKA)
info = struct('State', lkaState, 'Active', active, 'Authority', authority, ...
    'ControllerSelect', double(LKA.ControllerSelect), 'CurvatureReq', kReq, ...
    'CurvaturePP', kPP, 'CurvatureStanley', kSt, 'CurvatureMPC', kMpc, 'CurvatureFF', kFF, ...
    'CurvatureCmd', kCmd, 'CurvatureLimit', kMax, 'Lookahead', Ld, 'TargetOffset', yT, ...
    'SteerReq', dReq, 'SteerCmd', dCmd, 'CurvatureOut', kOut, 'TurnRadius', R, ...
    'LatAccelCmd', ay, 'Saturated', sat, 'LdwLeft', ldwL, 'LdwRight', ldwR, ...
    'DlcLeft', dlcL, 'DlcRight', dlcR, 'TlcLeft', tlcL, 'TlcRight', tlcR);

== matlab function LKA_Controller/Lane Perception/Lane Centre Estimation ==
  data: sensor input Bus: LaneSensorBus; z output; validL input; validR input; laneWidth input; zValid output; noiseScale output; numBoundaries output
function [z, zValid, noiseScale, numBoundaries] = fcn(sensor, validL, validR, laneWidth)
% Strength-weighted fusion of both boundaries into one lane-centre measurement
[z, zValid, noiseScale, numBoundaries] = lka_estimate_lane_center(sensor.Left, sensor.Right, validL, validR, laneWidth);

== matlab function LKA_Controller/Lane Perception/Boundary Validation ==
  data: sensor input Bus: LaneSensorBus; validL output boolean size=1; prevOffL input; prevOffR input; prevValidL input; prevValidR input; validR output boolean size=1; widthMeas output double size=1; widthValid output boolean size=1; offL output double size=1; offR output double size=1; LKA parameter
function [validL, validR, widthMeas, widthValid, offL, offR] = fcn(sensor, prevOffL, prevOffR, prevValidL, prevValidR, LKA)
% Plausibility gating of the detected boundaries (see lka_validate_boundaries.m)
[validL, validR, widthMeas, widthValid] = lka_validate_boundaries(sensor.Left, sensor.Right, ...
    prevOffL, prevOffR, prevValidL, prevValidR, LKA.Val, LKA.Lane);
validL = validL && sensor.FrameValid;
validR = validR && sensor.FrameValid;
offL = prevOffL; offR = prevOffR;
if validL, offL = sensor.Left.LateralOffset; end
if validR, offR = sensor.Right.LateralOffset; end

== matlab function LKA_Controller/Lane Perception/Lane State Tracker (Kalman) ==
  data: xPrev input; x output double size=[4 1]; PPrev input; stPrev input; z input; zValid input; noiseScale input; v input; yawRate input; P output double size=[4 4]; st output double size=[3 1]; quality output double size=1; LKA parameter
function [x, P, st, quality] = fcn(xPrev, PPrev, stPrev, z, zValid, noiseScale, v, yawRate, LKA)
% Kalman filter on [offset; heading; curvature; curvature rate] of the lane centre,
% predicted with vehicle speed and yaw rate (see lka_lane_tracker_step.m)
[x, P, st, quality] = lka_lane_tracker_step(xPrev, PPrev, stPrev, z, zValid, noiseScale, v, yawRate, LKA.Ts, LKA.KF);

== matlab function LKA_Controller/Lane Perception/Latency Compensation and Packing ==
  data: x input; est output Bus: LaneEstimateBus; laneWidth input; quality input; st input; zValid input; numBoundaries input; v input; yawRate input; LKA parameter
function est = fcn(x, laneWidth, quality, st, zValid, numBoundaries, v, yawRate, LKA)
% Detector frames are LKA.KF.LatencyComp old: move the estimate to the current time
xc = lka_lane_predict(x, v, yawRate, LKA.KF.LatencyComp);
est = struct('CenterOffset', xc(1), 'HeadingAngle', xc(2), 'Curvature', xc(3), ...
    'CurvatureDerivative', xc(4), 'LaneWidth', laneWidth, 'Quality', quality, ...
    'CoastTime', st(2), 'NumBoundaries', numBoundaries, 'MeasValid', zValid);

== stateflow chart LKA_Controller/LKA Supervisor/LKA Mode Logic ==
  settings: updateMethod=DISCRETE  sampleTime=LKA.Ts  description=LKA mode logic. OFF <-> ON by enable. Inside ON: STANDBY until speed and lane ok; ACTIVE steers; DEGRADED keeps steering on the tracker prediction while the lane is lost; TAKEOVER (no steering) when the lane is lost longer than LKA.Sup.CoastMax.
  state ON
    state STANDBY
      entry:
      lkaState = uint8(1);
      active = false;
    state ACTIVE
      entry:
      lkaState = uint8(2);
      active = true;
    state TAKEOVER
      entry:
      lkaState = uint8(4);
      active = false;
    state DEGRADED
      entry:
      lkaState = uint8(3);
      active = true;
    (default) -> STANDBY
    STANDBY -> ACTIVE : [speedOk && laneOk]
    ACTIVE -> STANDBY [order 1] : [~speedOk]
    TAKEOVER -> STANDBY : after(2,sec)[laneOk]
    DEGRADED -> STANDBY [order 2] : [~speedOk]
    DEGRADED -> ACTIVE [order 1] : [laneOk]
    ACTIVE -> DEGRADED [order 2] : [~laneOk]
    DEGRADED -> TAKEOVER [order 3] : [coastExceeded]
  state OFF
    entry:
    lkaState = uint8(0);
    active = false;
  OFF -> ON : [enable]
  (default) -> OFF
  ON -> OFF : [~enable]
  data: enable input boolean; speedOk input boolean; laneOk input boolean; coastExceeded input boolean; lkaState output uint8; active output boolean
